simulink model "FPGA_Compatible_FirstOrderADRC"  (R2026a)
settings: Solver=FixedStepDiscrete  StopTime=0.06  FixedStep=5e-9
undefined symbols (not defined in the file): ADC_Offset, adc_volts_per_count, alpha_iqd, alpha_s, beta_iqd, beta_s, biq, bs, electricalRadiansPerCount, gam_iqd, gam_s, Iq_limit, k1_iqd, k1_s, K_omega, KPth, mechanicalRadiansPerCount, PWMVoltage, theta_ref, Ts_current, Ts_sim, Ts_velocity
libraries: dspsigops x3, simulink x2, mcbeeMathTransformLib x2, hdlsllib x1
settings Model: DataTypeOverride=Off  Creator=mike  LastModifiedBy=Drew
settings OptimizationCC: ConditionallyExecuteInputs=off  InheritOutputTypeSmallerThanSingle=on
settings DebuggingCC: ArtificialAlgebraicLoopMsg=error  SingleTaskRateTransMsg=error  ParameterPrecisionLossMsg=none
settings HardwareCC: ProdHWDeviceType=ASIC/FPGA->ASIC/FPGA  TargetBitPerPointer=64.0  TargetBitPerSizeT=64.0  TargetBitPerPtrDiffT=64.0  TargetLongLongMode=on  TargetIntDivRoundTo=Zero  TargetEndianess=LittleEndian  TargetWordSize=64.0  TargetHWDeviceType=Custom Processor->MATLAB Host Computer  ProdEqTarget=off

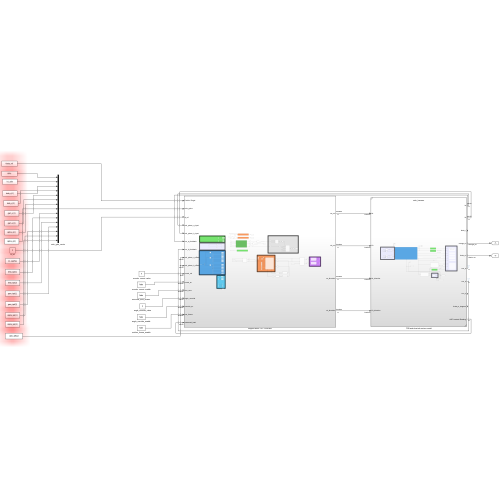
[thumbnail: Simulink's stored preview of the top-level diagram]
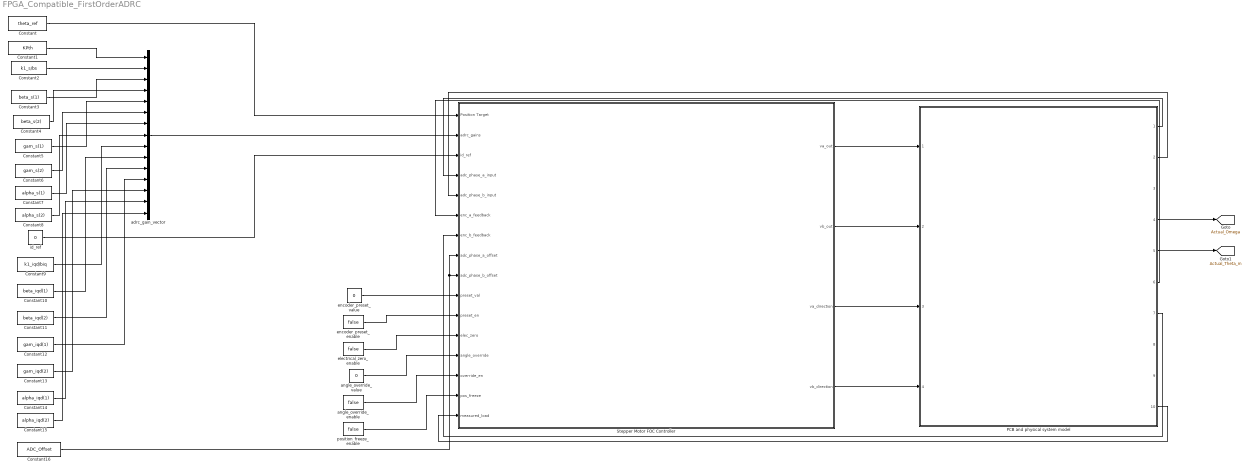
== system FPGA_Compatible_FirstOrderADRC ==
  Constant : Constant  Value=theta_ref  OutDataTypeStr=PosType  SampleTime=-1
  Constant1 : Constant  Value=KPth  OutDataTypeStr=ParamType
  Constant10 : Constant  Value=beta_iqd(1)  OutDataTypeStr=ParamType
  Constant11 : Constant  Value=beta_iqd(2)  OutDataTypeStr=ParamType
  Constant12 : Constant  Value=gam_iqd(1)  OutDataTypeStr=ParamType
  Constant13 : Constant  Value=gam_iqd(2)  OutDataTypeStr=ParamType
  Constant14 : Constant  Value=alpha_iqd(1)  OutDataTypeStr=ParamType
  Constant15 : Constant  Value=alpha_iqd(2)  OutDataTypeStr=ParamType
  Constant16 : Constant  Value=ADC_Offset
  Constant2 : Constant  Value=k1_s/bs  OutDataTypeStr=ParamType
  Constant3 : Constant  Value=beta_s(1)  OutDataTypeStr=ParamType
  Constant4 : Constant  Value=beta_s(2)  OutDataTypeStr=ParamType
  Constant5 : Constant  Value=gam_s(1)  OutDataTypeStr=ParamType
  Constant6 : Constant  Value=gam_s(2)  OutDataTypeStr=ParamType
  Constant7 : Constant  Value=alpha_s(1)  OutDataTypeStr=ParamType
  Constant8 : Constant  Value=alpha_s(2)  OutDataTypeStr=ParamType
  Constant9 : Constant  Value=k1_iqd/biq  OutDataTypeStr=ParamType
  PCB and physical system model : Subsystem  ReferencedSubsystem=adrc_harness
  Stepper Motor FOC Controller : Subsystem
  adrc_gain_vector : Mux  Inputs=15
  angle_override_enable : Constant  Value=false  OutDataTypeStr=boolean
  angle_override_value : Constant  Value=0  OutDataTypeStr=uint16
  electrical_zero_enable : Constant  Value=false  OutDataTypeStr=boolean
  encoder_preset_enable : Constant  Value=false  OutDataTypeStr=boolean
  encoder_preset_value : Constant  Value=0  OutDataTypeStr=fixdt(1,32,0)
  id_ref : Constant  Value=0  OutDataTypeStr=ParamType  SampleTime=-1
  position_freeze_enable : Constant  Value=false  OutDataTypeStr=boolean
  tag scope: Actual_Omega=global, Actual_Theta_m=global
  wires:
  Constant/1 -> Stepper Motor FOC Controller/1(Position Target)
  id_ref/1 -> Stepper Motor FOC Controller/3(id_ref)
  Stepper Motor FOC Controller/1(va_out) -> PCB and physical system model/1
  Stepper Motor FOC Controller/2(vb_out) -> PCB and physical system model/2
  PCB and physical system model/7 -> Stepper Motor FOC Controller/7(enc_b_feedback)
  PCB and physical system model/6 -> Stepper Motor FOC Controller/6(enc_a_feedback)
  PCB and physical system model/1 -> Stepper Motor FOC Controller/4(adc_phase_a_input)
  PCB and physical system model/2 -> Stepper Motor FOC Controller/5(adc_phase_b_input)
  PCB and physical system model/5 -> [Actual_Theta_m]
  Constant16/1 -> Stepper Motor FOC Controller/8(adc_phase_a_offset), Stepper Motor FOC Controller/9(adc_phase_b_offset)
  Stepper Motor FOC Controller/3(va_direction) -> PCB and physical system model/3
  Stepper Motor FOC Controller/4(vb_direction) -> PCB and physical system model/4
  PCB and physical system model/4 -> [Actual_Omega]
  PCB and physical system model/10 -> Stepper Motor FOC Controller/16(measured_load)
  position_freeze_enable/1 -> Stepper Motor FOC Controller/15(pos_freeze)
  angle_override_enable/1 -> Stepper Motor FOC Controller/14(override_en)
  angle_override_value/1 -> Stepper Motor FOC Controller/13(angle_override)
  electrical_zero_enable/1 -> Stepper Motor FOC Controller/12(elec_zero)
  encoder_preset_enable/1 -> Stepper Motor FOC Controller/11(preset_en)
  encoder_preset_value/1 -> Stepper Motor FOC Controller/10(preset_val)
  adrc_gain_vector/1 -> Stepper Motor FOC Controller/2(adrc_gains)
  Constant15/1 -> adrc_gain_vector/15
  Constant14/1 -> adrc_gain_vector/14
  Constant13/1 -> adrc_gain_vector/13
  Constant12/1 -> adrc_gain_vector/12
  Constant11/1 -> adrc_gain_vector/11
  Constant10/1 -> adrc_gain_vector/10
  Constant9/1 -> adrc_gain_vector/9
  Constant8/1 -> adrc_gain_vector/8
  Constant7/1 -> adrc_gain_vector/7
  Constant6/1 -> adrc_gain_vector/6
  Constant5/1 -> adrc_gain_vector/5
  Constant4/1 -> adrc_gain_vector/4
  Constant3/1 -> adrc_gain_vector/3
  Constant2/1 -> adrc_gain_vector/2
  Constant1/1 -> adrc_gain_vector/1

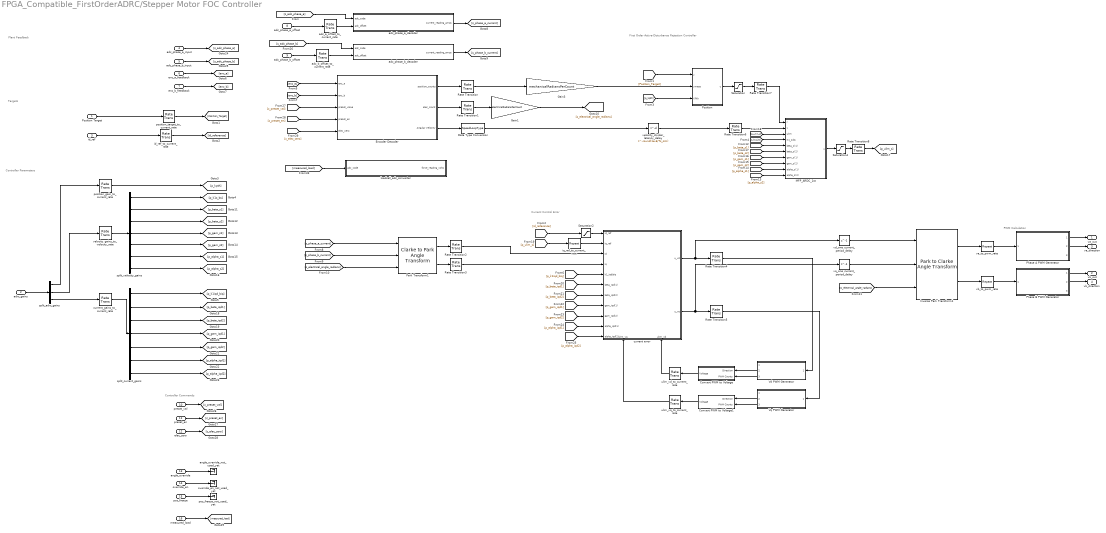
== system FPGA_Compatible_FirstOrderADRC/Stepper Motor FOC Controller ==
  note: PWM Calculation
  note: Current Control Error
  note: First Order Active-Disturbance Rejection Controller
  note: Controller Commands
  note: Controller Parameters
  note: Targets
  note: Plant Feedback
  Position Target : Inport  OutDataTypeStr=PosType  SampleTime=Ts_sim
  adrc_gains : Inport  Port=2  OutDataTypeStr=ParamType  PortDimensions=15  SampleTime=Ts_sim
  id_ref : Inport  Port=3  OutDataTypeStr=ParamType  SampleTime=Ts_sim
  adc_phase_a_input : Inport  Port=4
  adc_phase_b_input : Inport  Port=5
  enc_a_feedback : Inport  Port=6
  enc_b_feedback : Inport  Port=7
  adc_phase_a_offset : Inport  Port=8  OutDataTypeStr=uint16  SampleTime=Ts_sim
  adc_phase_b_offset : Inport  Port=9  OutDataTypeStr=uint16  SampleTime=Ts_sim
  preset_val : Inport  Port=10  OutDataTypeStr=fixdt(1,32,0)  SampleTime=Ts_sim
  preset_en : Inport  Port=11  OutDataTypeStr=boolean  SampleTime=Ts_sim
  elec_zero : Inport  Port=12  OutDataTypeStr=boolean  SampleTime=Ts_sim
  angle_override : Inport  Port=13  OutDataTypeStr=uint16  SampleTime=Ts_sim
  override_en : Inport  Port=14  OutDataTypeStr=boolean  SampleTime=Ts_sim
  pos_freeze : Inport  Port=15  OutDataTypeStr=boolean  SampleTime=Ts_sim
  measured_load : Inport  Port=16  OutDataTypeStr=uint16
  Convert PWM to Voltage : Subsystem
  Convert PWM to Voltage1 : Subsystem
  Data Type Conversion : DataTypeConversion  OutDataTypeStr=SpeedLoopType  RndMeth=Nearest
  Encoder Decoder : Subsystem
  Gain1 : Gain  Gain=electricalRadiansPerCount  OutDataTypeStr=PosType  SaturateOnIntegerOverflow=on
  Gain3 : Gain  Gain=mechanicalRadiansPerCount  OutDataTypeStr=PosType  SaturateOnIntegerOverflow=on
  Inverse Park Transform1 : mcbeeMathTransformLib/Park to Clarke Angle Transform  AxisAlignment=D-axis  UseWithEmbedded=on  PhaseInput=Two inputs  ThetaInput=Electrical position  AngleInput=Radians  N_points=1024
      settings: LibrarySourceBlock=mcbhdllib/Controls/Math Transforms/Inverse Park Transform
  MFP_ARDC_1st : Subsystem
  Park Transform1 : mcbeeMathTransformLib/Clarke to Park Angle Transform  AxisAlignment=D-axis  UseWithEmbedded=on  PhaseInput=Two inputs  ThetaInput=Electrical position  AngleInput=Radians  N_points=1024
      settings: LibrarySourceBlock=mcbhdllib/Controls/Math Transforms/Park Transform
  Phase A PWM Generator : Subsystem  ReferencedSubsystem=PWM_Generator
  Phase B PWM Generator : Subsystem  ReferencedSubsystem=PWM_Generator
  "Position " : Subsystem
  Rate Transition{,1..3} (4 alike) : RateTransition  OutPortSampleTime=2e-5
  Rate Transition4 : RateTransition  OutPortSampleTime=1e-7
  Rate Transition5 : RateTransition  OutPortSampleTime=1e-7
  Rate Transition6 : RateTransition  OutPortSampleTime=Ts_velocity
  Rate Transition7 : RateTransition  OutPortSampleTime=Ts_velocity
  Rate Transition8 : RateTransition  OutPortSampleTime=Ts_velocity
  Saturation : Saturate  UpperLimit=35.5  LowerLimit=-35.5
  Saturation2 : Saturate  UpperLimit=2.4  LowerLimit=-2.4  OutDataTypeStr=ParamType
  Saturation4 : Saturate  UpperLimit=Iq_limit  LowerLimit=-1*Iq_limit
  Vd PWM Generator : Subsystem  ReferencedSubsystem=PWM_Generator
  Vq PWM Generator : Subsystem  ReferencedSubsystem=PWM_Generator
  adc_a_offset_to_current_rate : RateTransition  OutPortSampleTime=Ts_current
  adc_b_offset_to_current_rate : RateTransition  OutPortSampleTime=Ts_current
  adc_phase_a_decoder : Subsystem
  adc_phase_b_decoder : Subsystem
  angle_override_not_used_yet : Terminator
  current error : Subsystem
      settings: PortSchema="{\"entries\":[{\"content\":{\"sides\":[{\"content\":{\"connectorIds\":[\"In1\",\"In2\",\"In3\",\"In4\",\"In5\",\"In6\",\"In7\",\"In8\",\"In9\",\"In10\",\"In11\"]},\"type\":\"ConnectorPlacement.EquallySpacedRectSide\",\"uuid\":\"1b67f1ba-d970-4a72-948b-8a645885f311\"},{\"content\":{\"connectorIds\":[\"Out1\",\"Out2\"],\"side\":\"RIGHT\"},\"type\":\"ConnectorPlacement.EquallySpacedRectSide\",\"uuid\":\"43bd9de9-c038-41d9-a38f-2b3bf68f84b7\"},{\"content\":{\"side\":\"TOP\"},\"type\":\"ConnectorPlacement.EquallySpacedRectSide\",\"uuid\":\"199b5c60-7e13-4435-9b33-d3faaa781c81\"},{\"content\":{\"connectorIds\":[\"In12\",\"In13\"],\"side\":\"BOTTOM\"},\"type\":\"ConnectorPlacement.EquallySpacedRectSide\",\"uuid\":\"8463aca4-e427-4dc0-a0b4-e373bcd68b49\"}]},\"type\":\"ConnectorPlacement.EquallySpacedConnector\",\"uuid\":\"7665834e-14df-482a-91d4-36c3c32286ac\"}],\"packageUris\":[\"http://schema.mathworks.com/mf0/Connector/R2020b\"],\"version\":\"1.0\"}"
  current_gains_to_current_rate : RateTransition  OutPortSampleTime=Ts_current
  id_ref_to_current_rate : RateTransition  OutPortSampleTime=Ts_current
  iq_ref_to_current_rate : dspsigops/Repeat  FactorSource=Dialog parameter  N=round(Ts_velocity/Ts_current)  Nmax=16  InputProcessing=Columns as channels (frame based)  RateOptions=Allow multirate processing  ic=0  mode=Unused parameter value
  loadcell_adc_converter : Subsystem
  override_en_not_used_yet : Terminator
  pos_freeze_not_used_yet : Terminator
  position_gain_to_current_rate : RateTransition  OutPortSampleTime=Ts_current
  position_target_to_current_rate : RateTransition  OutPortSampleTime=Ts_current
  split_adrc_gains : Demux  Outputs=[1 7 7]
  split_current_gains : Demux  Outputs=7
  split_velocity_gains : Demux  Outputs=7
  ulim_vd_to_current_rate : RateTransition  OutPortSampleTime=Ts_current
  ulim_vq_to_current_rate : RateTransition  OutPortSampleTime=Ts_current
  va_to_pwm_rate : dspsigops/Repeat  FactorSource=Dialog parameter  N=round(Ts_current/Ts_sim)  Nmax=16  InputProcessing=Columns as channels (frame based)  RateOptions=Allow multirate processing  ic=0  mode=Unused parameter value
  vb_to_pwm_rate : dspsigops/Repeat  FactorSource=Dialog parameter  N=round(Ts_current/Ts_sim)  Nmax=16  InputProcessing=Columns as channels (frame based)  RateOptions=Allow multirate processing  ic=0  mode=Unused parameter value
  vd_one_current_period_delay : Delay  DelayLength=1  InitialCondition=0
  velocity_divider_latency_delay : Delay  DelayLength=round(1e-6/Ts_sim)  InitialCondition=0
  velocity_gains_to_velocity_rate : RateTransition  OutPortSampleTime=Ts_velocity
  vq_one_current_period_delay : Delay  DelayLength=1  InitialCondition=0
  va_out : Outport  OutDataTypeStr=boolean
  vb_out : Outport  Port=2  OutDataTypeStr=boolean
  va_direction : Outport  Port=3  OutDataTypeStr=boolean
  vb_direction : Outport  Port=4  OutDataTypeStr=boolean
  wires:
  [Position_Target] -> "Position "/1(y)
  [p_kpth] -> "Position "/3(KPth)
  [p_k1s_bs] -> MFP_ARDC_1st/4(K1_s/bs)
  [p_k1iqd_biq] -> current error/5(k1_iqd/biq)
  enc_a_feedback/1 -> [enc_a]
  enc_b_feedback/1 -> [enc_b]
  adc_phase_a_decoder/1(current_reading_amps) -> [s_phase_a_current]
  adc_phase_b_decoder/1(current_reading_amps) -> [s_phase_b_current]
  [s_electrical_angle_radians] -> Park Transform1/3
  [s_electrical_angle_radians] -> Inverse Park Transform1/3
  [p_beta_s1] -> MFP_ARDC_1st/5(beta_s(1))
  [p_beta_s2] -> MFP_ARDC_1st/6(beta_s(2))
  [p_gam_s1] -> MFP_ARDC_1st/7(gam_s(1))
  [p_gam_s2] -> MFP_ARDC_1st/8(gam_s(2))
  [p_alpha_s1] -> MFP_ARDC_1st/9(alpha_s(1))
  [p_alpha_s2] -> MFP_ARDC_1st/10(alpha_s(2))
  MFP_ARDC_1st/1(u) -> Saturation4/1
  [p_ulim_s] -> MFP_ARDC_1st/3(ulim)
  [p_beta_iqd2] -> current error/7(beta_iqd(2))
  [p_beta_iqd1] -> current error/6(beta_iqd(1))
  [p_gam_iqd1] -> current error/8(gam_iqd(1))
  [p_gam_iqd2] -> current error/9(gam_iqd(2))
  [p_alpha_iqd1] -> current error/10(alpha_iqd(1))
  [p_alpha_iqd2] -> current error/11(alpha_iqd(2))
  adc_phase_a_input/1 -> [s_adc_phase_a]
  adc_phase_b_input/1 -> [s_adc_phase_b]
  [s_adc_phase_a] -> adc_phase_a_decoder/1(adc_code)
  [s_adc_phase_b] -> adc_phase_b_decoder/1(adc_code)
  elec_zero/1 -> [c_elec_zero]
  preset_en/1 -> [c_preset_en]
  preset_val/1 -> [c_preset_val]
  [id_reference] -> Saturation2/1
  Saturation2/1 -> current error/1(id_ref)
  Rate Transition/1 -> Gain3/1
  Rate Transition1/1 -> Gain1/1
  Gain1/1 -> [s_electrical_angle_radians]
  Gain3/1 -> "Position "/2(ymeas)
  Rate Transition2/1 -> current error/3(id)
  Rate Transition3/1 -> current error/4(iq)
  current error/1(u_vd) -> Rate Transition4/1, vd_one_current_period_delay/1
  Park Transform1/1 -> Rate Transition2/1
  Park Transform1/2 -> Rate Transition3/1
  "Position "/1(u) -> Saturation/1
  Phase A PWM Generator/1 -> va_out/1
  Phase A PWM Generator/2 -> va_direction/1
  Phase B PWM Generator/2 -> vb_direction/1
  Phase B PWM Generator/1 -> vb_out/1
  Rate Transition4/1 -> Vd PWM Generator/1
  Vd PWM Generator/2 -> Convert PWM to Voltage/1(Direction)
  Vd PWM Generator/3 -> Convert PWM to Voltage/2(PWM Counts)
  Vq PWM Generator/3 -> Convert PWM to Voltage1/2(PWM Counts)
  Vq PWM Generator/2 -> Convert PWM to Voltage1/1(Direction)
  measured_load/1 -> [measured_load]
  [measured_load] -> loadcell_adc_converter/1(adc_code)
  [enc_a] -> Encoder Decoder/1(enc_a)
  [enc_b] -> Encoder Decoder/2(enc_b)
  [c_preset_val] -> Encoder Decoder/3(preset_value)
  [c_preset_en] -> Encoder Decoder/4(preset_en)
  [c_elec_zero] -> Encoder Decoder/5(elec_zero)
  Encoder Decoder/1(position_counts) -> Rate Transition/1
  Encoder Decoder/2(elec_count) -> Rate Transition1/1
  Encoder Decoder/3(Angular Velocity) -> Data Type Conversion/1
  Saturation/1 -> Rate Transition7/1
  Rate Transition7/1 -> MFP_ARDC_1st/1(r)
  Rate Transition6/1 -> MFP_ARDC_1st/2(y)
  Saturation4/1 -> Rate Transition8/1
  Rate Transition8/1 -> [p_ulim_s]
  ulim_vq_to_current_rate/1 -> current error/12(ulim_vq)
  ulim_vd_to_current_rate/1 -> current error/13(ulim_vd)
  Convert PWM to Voltage/1(Voltage) -> ulim_vd_to_current_rate/1
  Convert PWM to Voltage1/1(Voltage) -> ulim_vq_to_current_rate/1
  iq_ref_to_current_rate/1 -> current error/2(iq_ref)
  [p_ulim_s] -> iq_ref_to_current_rate/1
  vb_to_pwm_rate/1 -> Phase B PWM Generator/1
  va_to_pwm_rate/1 -> Phase A PWM Generator/1
  vq_one_current_period_delay/1 -> Inverse Park Transform1/2
  vd_one_current_period_delay/1 -> Inverse Park Transform1/1
  Inverse Park Transform1/2 -> vb_to_pwm_rate/1
  Rate Transition5/1 -> Vq PWM Generator/1
  current error/2(u_vq) -> vq_one_current_period_delay/1, Rate Transition5/1
  Inverse Park Transform1/1 -> va_to_pwm_rate/1
  pos_freeze/1 -> pos_freeze_not_used_yet/1
  override_en/1 -> override_en_not_used_yet/1
  angle_override/1 -> angle_override_not_used_yet/1
  id_ref_to_current_rate/1 -> [id_reference]
  position_target_to_current_rate/1 -> [Position_Target]
  split_current_gains/7 -> [p_alpha_iqd2]
  split_current_gains/6 -> [p_alpha_iqd1]
  split_current_gains/5 -> [p_gam_iqd2]
  split_current_gains/4 -> [p_gam_iqd1]
  split_current_gains/3 -> [p_beta_iqd2]
  split_current_gains/2 -> [p_beta_iqd1]
  split_current_gains/1 -> [p_k1iqd_biq]
  current_gains_to_current_rate/1 -> split_current_gains/1
  split_adrc_gains/3 -> current_gains_to_current_rate/1
  split_velocity_gains/7 -> [p_alpha_s2]
  split_velocity_gains/6 -> [p_alpha_s1]
  split_velocity_gains/5 -> [p_gam_s2]
  split_velocity_gains/4 -> [p_gam_s1]
  split_velocity_gains/3 -> [p_beta_s2]
  split_velocity_gains/2 -> [p_beta_s1]
  split_velocity_gains/1 -> [p_k1s_bs]
  velocity_gains_to_velocity_rate/1 -> split_velocity_gains/1
  position_gain_to_current_rate/1 -> [p_kpth]
  adrc_gains/1 -> split_adrc_gains/1
  split_adrc_gains/1 -> position_gain_to_current_rate/1
  split_adrc_gains/2 -> velocity_gains_to_velocity_rate/1
  id_ref/1 -> id_ref_to_current_rate/1
  Position Target/1 -> position_target_to_current_rate/1
  [s_phase_a_current] -> Park Transform1/1
  [s_phase_b_current] -> Park Transform1/2
  adc_b_offset_to_current_rate/1 -> adc_phase_b_decoder/2(adc_offset)
  adc_a_offset_to_current_rate/1 -> adc_phase_a_decoder/2(adc_offset)
  adc_phase_b_offset/1 -> adc_b_offset_to_current_rate/1
  adc_phase_a_offset/1 -> adc_a_offset_to_current_rate/1
  velocity_divider_latency_delay/1 -> Rate Transition6/1
  Data Type Conversion/1 -> velocity_divider_latency_delay/1

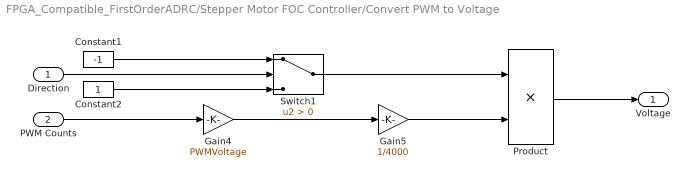
== system FPGA_Compatible_FirstOrderADRC/Stepper Motor FOC Controller/Convert PWM to Voltage ==
  Direction : Inport
  PWM Counts : Inport  Port=2
  Constant1 : Constant  Value=-1  OutDataTypeStr=fixdt(1,2,0)
  Constant2 : Constant  OutDataTypeStr=fixdt(1,2,0)
  Gain4 : Gain  Gain=PWMVoltage
  Gain5 : Gain  Gain=1/4000  OutDataTypeStr=ParamType
  Product : Product  OutDataTypeStr=ParamType
  Switch1 : Switch  Criteria=u2 > Threshold  SaturateOnIntegerOverflow=off  InputSameDT=off
  Voltage : Outport
  wires:
  Gain4/1 -> Gain5/1
  Gain5/1 -> Product/2
  Switch1/1 -> Product/1
  Constant1/1 -> Switch1/1
  Constant2/1 -> Switch1/3
  PWM Counts/1 -> Gain4/1
  Direction/1 -> Switch1/2
  Product/1 -> Voltage/1

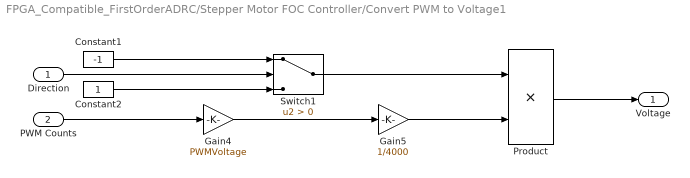
== system FPGA_Compatible_FirstOrderADRC/Stepper Motor FOC Controller/Convert PWM to Voltage1 ==
  Direction : Inport
  PWM Counts : Inport  Port=2
  Constant1 : Constant  Value=-1  OutDataTypeStr=fixdt(1,2,0)
  Constant2 : Constant  OutDataTypeStr=fixdt(1,2,0)
  Gain4 : Gain  Gain=PWMVoltage
  Gain5 : Gain  Gain=1/4000  OutDataTypeStr=ParamType
  Product : Product  OutDataTypeStr=ParamType
  Switch1 : Switch  Criteria=u2 > Threshold  SaturateOnIntegerOverflow=off  InputSameDT=off
  Voltage : Outport
  wires:
  Gain4/1 -> Gain5/1
  Gain5/1 -> Product/2
  Switch1/1 -> Product/1
  Constant1/1 -> Switch1/1
  Constant2/1 -> Switch1/3
  PWM Counts/1 -> Gain4/1
  Direction/1 -> Switch1/2
  Product/1 -> Voltage/1

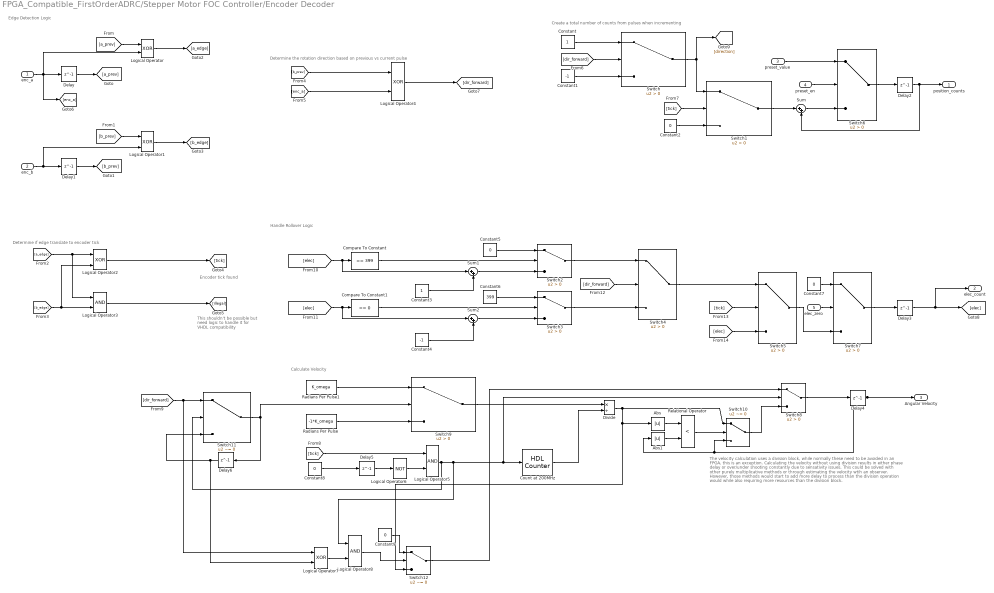
== system FPGA_Compatible_FirstOrderADRC/Stepper Motor FOC Controller/Encoder Decoder ==
  note: The velocity calculation uses a division block, while normally these need to be avoided in an FPGA, this is an exception. Calculating the velocity without using division results in either phase delay or over/under shooting constantly due to sensativity issues. This could be solved with other purely multiplicative methods or through estimating the velocity wtih an observer. However, those methods would start to add more delay to process than the division operation would while also requiring more resources than the division block.
  note: Calculate Velocity
  note: Handle Rollover Logic
  note: Create a total number of counts from pulses when incrementing
  note: Determine the rotation direction based on previous vs current pulse
  note: Encoder tick found
  note: Determine if edge translate to encoder tick
  note: Edge Detection Logic
  note: This shouldn't be possible but need logic to handle it for VHDL compatibility
  enc_a : Inport  OutDataTypeStr=boolean
  enc_b : Inport  Port=2  OutDataTypeStr=boolean
  preset_value : Inport  Port=3  OutDataTypeStr=fixdt(1,32,0)
  preset_en : Inport  Port=4  OutDataTypeStr=boolean
  elec_zero : Inport  Port=5  OutDataTypeStr=boolean
  Abs : Abs
  Abs1 : Abs
  Compare To Constant : simulink/Logic and Bit Operations/Compare To Constant  relop===  const=399  OutDataTypeStr=boolean
  Compare To Constant1 : simulink/Logic and Bit Operations/Compare To Constant  relop===  const=0  OutDataTypeStr=boolean
  Constant : Constant  OutDataTypeStr=int32
  Constant1 : Constant  Value=-1  OutDataTypeStr=int32
  Constant2 : Constant  Value=0  OutDataTypeStr=int32
  Constant3 : Constant  OutDataTypeStr=int32
  Constant4 : Constant  Value=-1  OutDataTypeStr=int32
  Constant5 : Constant  Value=0  OutDataTypeStr=int32
  Constant6 : Constant  Value=399  OutDataTypeStr=int32
  Constant7 : Constant  Value=0  OutDataTypeStr=int32
  Constant8 : Constant  Value=0  OutDataTypeStr=boolean
  Constant9 : Constant  Value=0  OutDataTypeStr=SpeedLoopType
  Count at 200MHz : hdlsllib/Sources/HDL Counter  CountType=Count limited  CountInit=1  CountStep=1  CountMax=199999999  CountFromType=Initial value  CountFrom=1  CountResetPort=on  CountLoadPort=off  CountEnbPort=off  CountDirPort=off  CountHitOutputPort=off  CountDataType=Unsigned  CountWordLen=32  CountFracLen=0  CountSampTime=5e-9
  Delay{,1..4} (5 alike) : Delay  DelayLength=1  InputProcessing=Columns as channels (frame based)  SampleTime=Ts_sim
  Delay5 : Delay  DelayLength=1  InitialCondition=1  SampleTime=Ts_sim
  Delay6 : Delay  DelayLength=1  SampleTime=Ts_sim
  Divide : Product  Inputs=*/  OutDataTypeStr=SpeedLoopType  RndMeth=Nearest  SaturateOnIntegerOverflow=on
  Logical Operator{,1..2,4,7} (5 alike) : Logic  Operator=XOR  AllPortsSameDT=off  OutDataTypeStr=boolean
  Logical Operator3 : Logic  AllPortsSameDT=off  OutDataTypeStr=boolean
  Logical Operator5 : Logic  AllPortsSameDT=off  OutDataTypeStr=boolean
  Logical Operator6 : Logic  Operator=NOT  AllPortsSameDT=off  OutDataTypeStr=boolean
  Logical Operator8 : Logic  AllPortsSameDT=off  OutDataTypeStr=boolean
  Radians Per Pulse : Constant  Value=-1*K_omega  OutDataTypeStr=VelType
  Radians Per Pulse1 : Constant  Value=K_omega  OutDataTypeStr=VelType
  Relational Operator : RelationalOperator  Operator=<  OutDataTypeStr=boolean  RndMeth=Simplest  InputSameDT=off
  Sum : Sum  Inputs=|++  OutDataTypeStr=int32  SaturateOnIntegerOverflow=on
  Sum1 : Sum  Inputs=|++  OutDataTypeStr=int32
  Sum2 : Sum  Inputs=|++  OutDataTypeStr=int32
  Switch{,1..5} (6 alike) : Switch  Criteria=u2 > Threshold  SaturateOnIntegerOverflow=off  InputSameDT=off
  Switch10 : Switch  Criteria=u2 ~= 0  OutDataTypeStr=SpeedLoopType  SaturateOnIntegerOverflow=off  InputSameDT=off
  Switch11 : Switch  Criteria=u2 ~= 0  OutDataTypeStr=boolean  SaturateOnIntegerOverflow=off  InputSameDT=off
  Switch12 : Switch  Criteria=u2 ~= 0  OutDataTypeStr=SpeedLoopType  SaturateOnIntegerOverflow=off  InputSameDT=off
  Switch6 : Switch  Criteria=u2 > Threshold  OutDataTypeStr=CountType  SaturateOnIntegerOverflow=off  InputSameDT=off
  Switch7 : Switch  Criteria=u2 > Threshold  OutDataTypeStr=CountType  SaturateOnIntegerOverflow=off  InputSameDT=off
  Switch8 : Switch  Criteria=u2 > Threshold  OutDataTypeStr=SpeedLoopType  SaturateOnIntegerOverflow=off  InputSameDT=off
  Switch9 : Switch  Criteria=u2 > Threshold  OutDataTypeStr=VelType  SaturateOnIntegerOverflow=off  InputSameDT=off
  position_counts : Outport  OutDataTypeStr=CountType
  elec_count : Outport  Port=2  OutDataTypeStr=CountType
  Angular Velocity : Outport  Port=3  OutDataTypeStr=SpeedLoopType
  wires:
  enc_b/1 -> Logical Operator1/2, Delay1/1
  enc_a/1 -> [enc_a], Logical Operator/2, Delay/1
  Delay/1 -> [a_prev]
  Delay1/1 -> [b_prev]
  [b_prev] -> Logical Operator1/1
  [a_prev] -> Logical Operator/1
  Logical Operator/1 -> [a_edge]
  Logical Operator1/1 -> [b_edge]
  [b_edge] -> Logical Operator3/2, Logical Operator2/2
  [a_edge] -> Logical Operator2/1, Logical Operator3/1
  Logical Operator2/1 -> [tick]
  Logical Operator3/1 -> [illegal]
  [b_prev] -> Logical Operator4/1
  [enc_a] -> Logical Operator4/2
  Logical Operator4/1 -> [dir_forward]
  Constant/1 -> Switch/1
  Constant1/1 -> Switch/3
  [dir_forward] -> Switch/2
  [tick] -> Switch1/2
  Constant2/1 -> Switch1/3
  Switch/1 -> Switch1/1, [direction]
  Switch1/1 -> Sum/1
  Delay2/1 -> Sum/2, position_counts/1
  Constant5/1 -> Switch2/1
  Compare To Constant1/1 -> Switch3/2
  Sum2/1 -> Switch3/3
  Sum1/1 -> Switch2/3
  Constant6/1 -> Switch3/1
  [elec] -> Sum2/1, Compare To Constant1/1
  [elec] -> Sum1/1, Compare To Constant/1
  Switch2/1 -> Switch4/1
  Constant3/1 -> Sum1/2
  Compare To Constant/1 -> Switch2/2
  Constant4/1 -> Sum2/2
  [dir_forward] -> Switch4/2
  Switch3/1 -> Switch4/3
  Switch4/1 -> Switch5/1
  [tick] -> Switch5/2
  [elec] -> Switch5/3
  Delay3/1 -> elec_count/1, [elec]
  Sum/1 -> Switch6/3
  Switch6/1 -> Delay2/1
  preset_en/1 -> Switch6/2
  preset_value/1 -> Switch6/1
  Constant7/1 -> Switch7/1
  elec_zero/1 -> Switch7/2
  Switch5/1 -> Switch7/3
  Switch7/1 -> Delay3/1
  Count at 200MHz/1 -> Divide/2
  Switch8/1 -> Delay4/1
  Delay4/1 -> Switch10/3, Abs1/1, Angular Velocity/1
  Switch9/1 -> Divide/1
  Radians Per Pulse/1 -> Switch9/3
  Radians Per Pulse1/1 -> Switch9/1
  Divide/1 -> Switch12/3, Abs/1, Switch10/1
  [dir_forward] -> Logical Operator7/1, Switch11/1
  [tick] -> Logical Operator5/1
  Abs1/1 -> Relational Operator/2
  Abs/1 -> Relational Operator/1
  Switch10/1 -> Switch8/3
  Relational Operator/1 -> Switch10/2
  Logical Operator5/1 -> Switch11/2, Logical Operator8/1, Switch8/2, Count at 200MHz/1
  Delay5/1 -> Logical Operator6/1
  Constant8/1 -> Delay5/1
  Logical Operator6/1 -> Logical Operator5/2
  Switch11/1 -> Delay6/1, Switch9/2
  Delay6/1 -> Logical Operator7/2, Switch11/3
  Logical Operator7/1 -> Logical Operator8/2
  Constant9/1 -> Switch12/1
  Logical Operator8/1 -> Switch12/2
  Switch12/1 -> Switch8/1

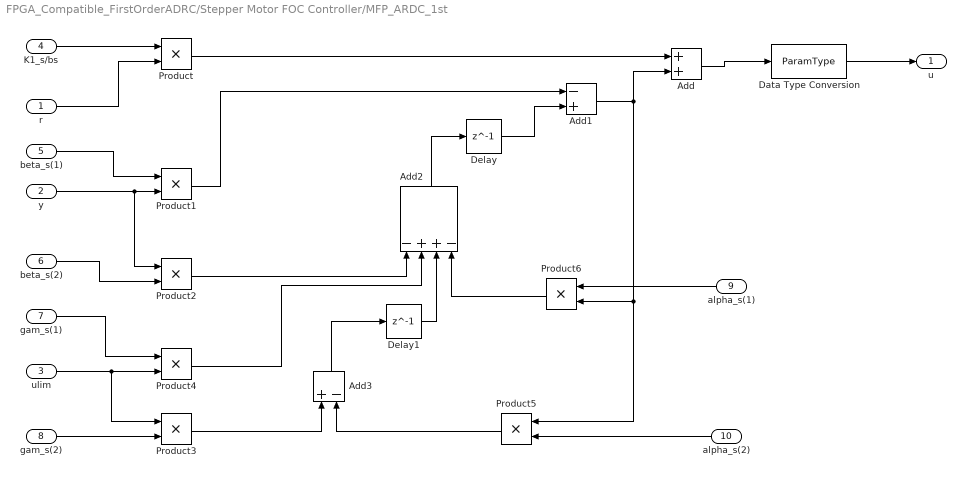
== system FPGA_Compatible_FirstOrderADRC/Stepper Motor FOC Controller/MFP_ARDC_1st ==
  r : Inport  OutDataTypeStr=PosType
  y : Inport  Port=2  OutDataTypeStr=PosType
  ulim : Inport  Port=3  OutDataTypeStr=ParamType
  K1_s/bs : Inport  Port=4  OutDataTypeStr=ParamType
  beta_s(1) : Inport  Port=5  OutDataTypeStr=ParamType
  beta_s(2) : Inport  Port=6  OutDataTypeStr=ParamType
  gam_s(1) : Inport  Port=7  OutDataTypeStr=ParamType
  gam_s(2) : Inport  Port=8  OutDataTypeStr=ParamType
  alpha_s(1) : Inport  Port=9  OutDataTypeStr=ParamType
  alpha_s(2) : Inport  Port=10  OutDataTypeStr=ParamType
  Add : Sum  OutDataTypeStr=SpeedLoopType  SaturateOnIntegerOverflow=on
  Add1 : Sum  Inputs=-+  OutDataTypeStr=SpeedLoopType  SaturateOnIntegerOverflow=on
  Add2 : Sum  Inputs=-++-  OutDataTypeStr=SpeedLoopType  SaturateOnIntegerOverflow=on
  Add3 : Sum  Inputs=+-  OutDataTypeStr=SpeedLoopType  SaturateOnIntegerOverflow=on
  Data Type Conversion : DataTypeConversion  OutDataTypeStr=ParamType  RndMeth=Floor
  Delay : Delay  DelayLength=1  InitialCondition=0  SampleTime=Ts_velocity
  Delay1 : Delay  DelayLength=1  InitialCondition=0  SampleTime=Ts_velocity
  Product{,1..6} (7 alike) : Product  OutDataTypeStr=SpeedLoopType  SaturateOnIntegerOverflow=on
  u : Outport  OutDataTypeStr=ParamType
  wires:
  Add/1 -> Data Type Conversion/1
  Add3/1 -> Delay1/1
  Product4/1 -> Add2/2
  Product6/1 -> Add2/4
  Add1/1 -> Product5/1, Product6/2, Add/2
  Add2/1 -> Delay/1
  r/1 -> Product/2
  Delay1/1 -> Add2/3
  Product3/1 -> Add3/1
  ulim/1 -> Product3/1, Product4/2
  Product2/1 -> Add2/1
  Product5/1 -> Add3/2
  Delay/1 -> Add1/2
  Product1/1 -> Add1/1
  y/1 -> Product2/1, Product1/2
  K1_s/bs/1 -> Product/1
  Product/1 -> Add/1
  beta_s(1)/1 -> Product1/1
  beta_s(2)/1 -> Product2/2
  gam_s(1)/1 -> Product4/1
  gam_s(2)/1 -> Product3/2
  alpha_s(2)/1 -> Product5/2
  alpha_s(1)/1 -> Product6/1
  Data Type Conversion/1 -> u/1

== system FPGA_Compatible_FirstOrderADRC/Stepper Motor FOC Controller/Position  ==
  y : Inport  OutDataTypeStr=PosType
  ymeas : Inport  Port=2  OutDataTypeStr=PosType
  KPth : Inport  Port=3  OutDataTypeStr=ParamType
  Product : Product  OutDataTypeStr=PosType  SaturateOnIntegerOverflow=on
  Sum : Sum  Inputs=|+-  OutDataTypeStr=PosType  SaturateOnIntegerOverflow=on
  u : Outport  OutDataTypeStr=PosType
  wires:
  y/1 -> Sum/1
  ymeas/1 -> Sum/2
  Sum/1 -> Product/2
  Product/1 -> u/1
  KPth/1 -> Product/1

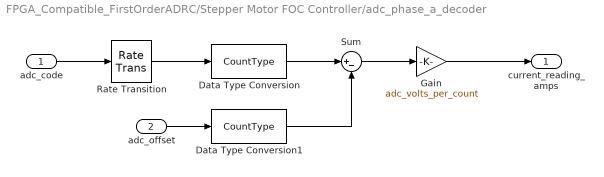
== system FPGA_Compatible_FirstOrderADRC/Stepper Motor FOC Controller/adc_phase_a_decoder ==
  adc_code : Inport  OutMin=[0]  OutDataTypeStr=uint16
  adc_offset : Inport  Port=2  OutDataTypeStr=uint16
  Data Type Conversion : DataTypeConversion  OutDataTypeStr=CountType  RndMeth=Round
  Data Type Conversion1 : DataTypeConversion  OutDataTypeStr=CountType  RndMeth=Round
  Gain : Gain  Gain=adc_volts_per_count  ParamDataTypeStr=fixdt(0,32,38)  OutDataTypeStr=ParamType  RndMeth=Round  SaturateOnIntegerOverflow=on
  Rate Transition : RateTransition  OutPortSampleTime=2e-5
  Sum : Sum  Inputs=|+-  OutDataTypeStr=CountType  AccumDataTypeStr=CountType  RndMeth=Round  SaturateOnIntegerOverflow=on
  current_reading_amps : Outport  OutDataTypeStr=ParamType
  wires:
  adc_offset/1 -> Data Type Conversion1/1
  Data Type Conversion1/1 -> Sum/2
  Data Type Conversion/1 -> Sum/1
  Sum/1 -> Gain/1
  Gain/1 -> current_reading_amps/1
  adc_code/1 -> Rate Transition/1
  Rate Transition/1 -> Data Type Conversion/1

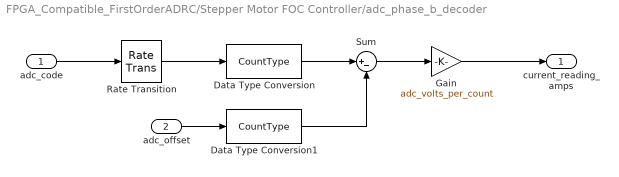
== system FPGA_Compatible_FirstOrderADRC/Stepper Motor FOC Controller/adc_phase_b_decoder ==
  adc_code : Inport  OutMin=[0]  OutDataTypeStr=uint16
  adc_offset : Inport  Port=2  OutDataTypeStr=uint16
  Data Type Conversion : DataTypeConversion  OutDataTypeStr=CountType  RndMeth=Round
  Data Type Conversion1 : DataTypeConversion  OutDataTypeStr=CountType  RndMeth=Round
  Gain : Gain  Gain=adc_volts_per_count  ParamDataTypeStr=fixdt(0,32,38)  OutDataTypeStr=ParamType  RndMeth=Round  SaturateOnIntegerOverflow=on
  Rate Transition : RateTransition  OutPortSampleTime=2e-5
  Sum : Sum  Inputs=|+-  OutDataTypeStr=CountType  AccumDataTypeStr=CountType  RndMeth=Round  SaturateOnIntegerOverflow=on
  current_reading_amps : Outport  OutDataTypeStr=ParamType
  wires:
  adc_offset/1 -> Data Type Conversion1/1
  Data Type Conversion1/1 -> Sum/2
  Data Type Conversion/1 -> Sum/1
  Sum/1 -> Gain/1
  Gain/1 -> current_reading_amps/1
  Rate Transition/1 -> Data Type Conversion/1
  adc_code/1 -> Rate Transition/1

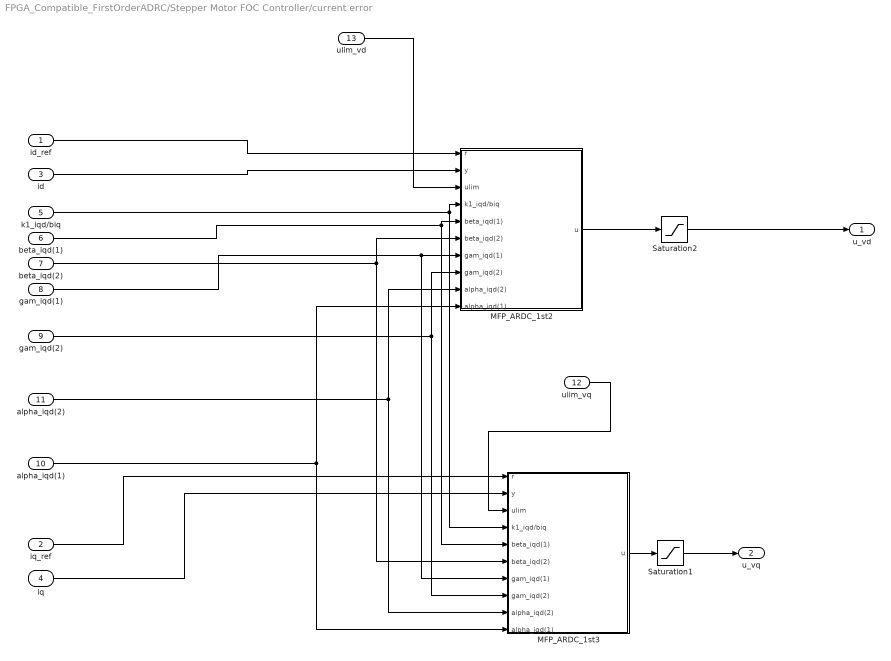
== system FPGA_Compatible_FirstOrderADRC/Stepper Motor FOC Controller/current error ==
  id_ref : Inport  OutDataTypeStr=ParamType
  iq_ref : Inport  Port=2  OutDataTypeStr=ParamType
  id : Inport  Port=3  OutDataTypeStr=ParamType
  iq : Inport  Port=4  OutDataTypeStr=ParamType
  k1_iqd/biq : Inport  Port=5  OutDataTypeStr=ParamType
  beta_iqd(1) : Inport  Port=6  OutDataTypeStr=ParamType
  beta_iqd(2) : Inport  Port=7  OutDataTypeStr=ParamType
  gam_iqd(1) : Inport  Port=8  OutDataTypeStr=ParamType
  gam_iqd(2) : Inport  Port=9  OutDataTypeStr=ParamType
  alpha_iqd(1) : Inport  Port=10  OutDataTypeStr=ParamType
  alpha_iqd(2) : Inport  Port=11  OutDataTypeStr=ParamType
  ulim_vq : Inport  Port=12
  ulim_vd : Inport  Port=13
  MFP_ARDC_1st2 : Subsystem
  MFP_ARDC_1st3 : Subsystem
  Saturation1 : Saturate  UpperLimit=PWMVoltage  LowerLimit=-1*PWMVoltage  OutDataTypeStr=ParamType
  Saturation2 : Saturate  UpperLimit=PWMVoltage  LowerLimit=-1*PWMVoltage  OutDataTypeStr=ParamType
  u_vd : Outport  OutDataTypeStr=ParamType
  u_vq : Outport  Port=2  OutDataTypeStr=ParamType
  wires:
  iq_ref/1 -> MFP_ARDC_1st3/1(r)
  iq/1 -> MFP_ARDC_1st3/2(y)
  Saturation1/1 -> u_vq/1
  MFP_ARDC_1st3/1(u) -> Saturation1/1
  id/1 -> MFP_ARDC_1st2/2(y)
  id_ref/1 -> MFP_ARDC_1st2/1(r)
  MFP_ARDC_1st2/1(u) -> Saturation2/1
  Saturation2/1 -> u_vd/1
  k1_iqd/biq/1 -> MFP_ARDC_1st2/4(k1_iqd/biq), MFP_ARDC_1st3/4(k1_iqd/biq)
  beta_iqd(1)/1 -> MFP_ARDC_1st2/5(beta_iqd(1)), MFP_ARDC_1st3/5(beta_iqd(1))
  beta_iqd(2)/1 -> MFP_ARDC_1st3/6(beta_iqd(2)), MFP_ARDC_1st2/6(beta_iqd(2))
  gam_iqd(1)/1 -> MFP_ARDC_1st2/7(gam_iqd(1)), MFP_ARDC_1st3/7(gam_iqd(1))
  gam_iqd(2)/1 -> MFP_ARDC_1st2/8(gam_iqd(2)), MFP_ARDC_1st3/8(gam_iqd(2))
  alpha_iqd(2)/1 -> MFP_ARDC_1st2/9(alpha_iqd(2)), MFP_ARDC_1st3/9(alpha_iqd(2))
  alpha_iqd(1)/1 -> MFP_ARDC_1st2/10(alpha_iqd(1)), MFP_ARDC_1st3/10(alpha_iqd(1))
  ulim_vd/1 -> MFP_ARDC_1st2/3(ulim)
  ulim_vq/1 -> MFP_ARDC_1st3/3(ulim)

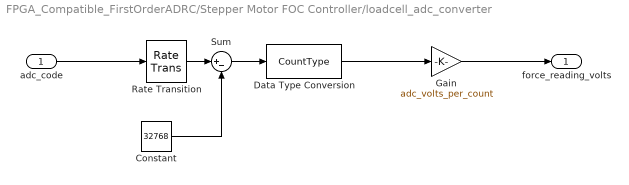
== system FPGA_Compatible_FirstOrderADRC/Stepper Motor FOC Controller/loadcell_adc_converter ==
  adc_code : Inport  OutMin=[0]  OutDataTypeStr=uint16
  Constant : Constant  Value=32768  OutDataTypeStr=uint16
  Data Type Conversion : DataTypeConversion  OutDataTypeStr=CountType  RndMeth=Floor
  Gain : Gain  Gain=adc_volts_per_count  ParamDataTypeStr=fixdt(0,32,38)  OutDataTypeStr=ParamType  RndMeth=Nearest  SaturateOnIntegerOverflow=on
  Rate Transition : RateTransition  OutPortSampleTime=2e-5
  Sum : Sum  Inputs=|+-  OutDataTypeStr=CountType  SaturateOnIntegerOverflow=on
  force_reading_volts : Outport  OutDataTypeStr=ParamType
  wires:
  Gain/1 -> force_reading_volts/1
  adc_code/1 -> Rate Transition/1
  Data Type Conversion/1 -> Gain/1
  Rate Transition/1 -> Sum/1
  Sum/1 -> Data Type Conversion/1
  Constant/1 -> Sum/2

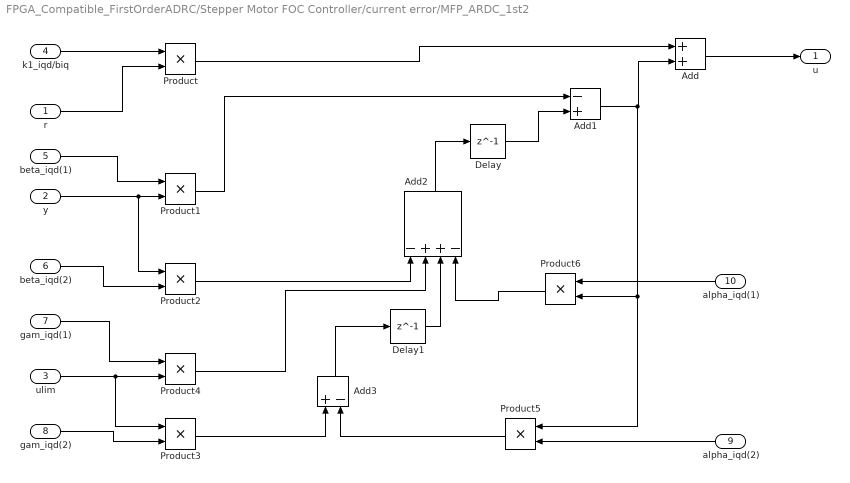
== system FPGA_Compatible_FirstOrderADRC/Stepper Motor FOC Controller/current error/MFP_ARDC_1st2 ==
  r : Inport
  y : Inport  Port=2
  ulim : Inport  Port=3
  k1_iqd/biq : Inport  Port=4
  beta_iqd(1) : Inport  Port=5
  beta_iqd(2) : Inport  Port=6
  gam_iqd(1) : Inport  Port=7
  gam_iqd(2) : Inport  Port=8
  alpha_iqd(2) : Inport  Port=9
  alpha_iqd(1) : Inport  Port=10
  Add : Sum  OutDataTypeStr=CurrLoopType  SaturateOnIntegerOverflow=on
  Add1 : Sum  Inputs=-+  OutDataTypeStr=CurrLoopType  SaturateOnIntegerOverflow=on
  Add2 : Sum  Inputs=-++-  OutDataTypeStr=CurrLoopType  SaturateOnIntegerOverflow=on
  Add3 : Sum  Inputs=+-  OutDataTypeStr=CurrLoopType  SaturateOnIntegerOverflow=on
  Delay : Delay  DelayLength=1  InitialCondition=0  SampleTime=Ts_current
  Delay1 : Delay  DelayLength=1  InitialCondition=0  SampleTime=Ts_current
  Product{,1..6} (7 alike) : Product  OutDataTypeStr=CurrLoopType  SaturateOnIntegerOverflow=on
  u : Outport
  wires:
  Add/1 -> u/1
  Add3/1 -> Delay1/1
  Product4/1 -> Add2/2
  Product6/1 -> Add2/4
  Add1/1 -> Product5/1, Product6/2, Add/2
  Add2/1 -> Delay/1
  r/1 -> Product/2
  Delay1/1 -> Add2/3
  Product3/1 -> Add3/1
  ulim/1 -> Product3/1, Product4/2
  Product2/1 -> Add2/1
  Product5/1 -> Add3/2
  Delay/1 -> Add1/2
  Product1/1 -> Add1/1
  y/1 -> Product2/1, Product1/2
  k1_iqd/biq/1 -> Product/1
  Product/1 -> Add/1
  beta_iqd(1)/1 -> Product1/1
  beta_iqd(2)/1 -> Product2/2
  gam_iqd(1)/1 -> Product4/1
  gam_iqd(2)/1 -> Product3/2
  alpha_iqd(2)/1 -> Product5/2
  alpha_iqd(1)/1 -> Product6/1

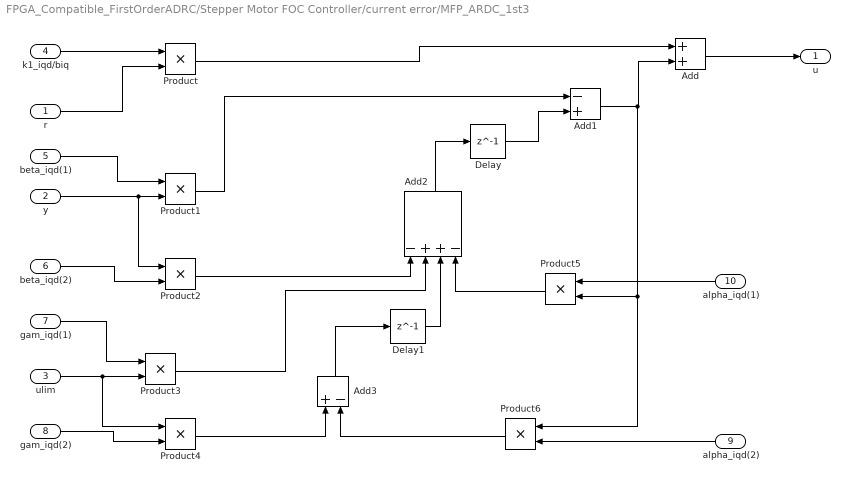
== system FPGA_Compatible_FirstOrderADRC/Stepper Motor FOC Controller/current error/MFP_ARDC_1st3 ==
  r : Inport
  y : Inport  Port=2
  ulim : Inport  Port=3
  k1_iqd/biq : Inport  Port=4
  beta_iqd(1) : Inport  Port=5
  beta_iqd(2) : Inport  Port=6
  gam_iqd(1) : Inport  Port=7
  gam_iqd(2) : Inport  Port=8
  alpha_iqd(2) : Inport  Port=9
  alpha_iqd(1) : Inport  Port=10
  Add : Sum  OutDataTypeStr=CurrLoopType  SaturateOnIntegerOverflow=on
  Add1 : Sum  Inputs=-+  OutDataTypeStr=CurrLoopType  SaturateOnIntegerOverflow=on
  Add2 : Sum  Inputs=-++-  OutDataTypeStr=CurrLoopType  SaturateOnIntegerOverflow=on
  Add3 : Sum  Inputs=+-  OutDataTypeStr=CurrLoopType  SaturateOnIntegerOverflow=on
  Delay : Delay  DelayLength=1  InitialCondition=0  SampleTime=Ts_current
  Delay1 : Delay  DelayLength=1  InitialCondition=0  SampleTime=Ts_current
  Product{,1..6} (7 alike) : Product  OutDataTypeStr=CurrLoopType  SaturateOnIntegerOverflow=on
  u : Outport
  wires:
  Add/1 -> u/1
  Add3/1 -> Delay1/1
  Product3/1 -> Add2/2
  Product5/1 -> Add2/4
  Add1/1 -> Product6/1, Product5/2, Add/2
  Add2/1 -> Delay/1
  r/1 -> Product/2
  Delay1/1 -> Add2/3
  Product4/1 -> Add3/1
  ulim/1 -> Product4/1, Product3/2
  Product2/1 -> Add2/1
  Product6/1 -> Add3/2
  Delay/1 -> Add1/2
  Product1/1 -> Add1/1
  y/1 -> Product2/1, Product1/2
  k1_iqd/biq/1 -> Product/1
  Product/1 -> Add/1
  beta_iqd(1)/1 -> Product1/1
  beta_iqd(2)/1 -> Product2/2
  gam_iqd(1)/1 -> Product3/1
  gam_iqd(2)/1 -> Product4/2
  alpha_iqd(2)/1 -> Product6/2
  alpha_iqd(1)/1 -> Product5/1
